simulink model "generic_IVS"  (R2024a)
settings: Solver=FixedStepDiscrete  StartTime=0.0  StopTime=inf  FixedStep=0.001  RelTol=1e-3  EnableMultiTasking=on
libraries: simulink x1, CarMaker4SL x1
(part 1 of 2)
settings Model: Creator=IPG  LastModifiedBy=User
settings SolverCC: AlgebraicLoopSolver=TrustRegion
settings DataIOCC: LimitDataPoints=on  SaveFormat=Array  SignalLoggingSaveFormat=ModelDataLogs  ReturnWorkspaceOutputs=off  SignalLoggingName=sigsOut
settings OptimizationCC: BooleanDataType=off  ReuseModelBlockBuffer=off  ExpressionDepthLimit=2147483647  InitFltsAndDblsToZero=on  LifeSpan=inf
settings DebuggingCC: SaveWithParameterizedLinksMsg=none  UnderspecifiedInitializationDetection=Classic  MergeDetectMultiDrivingBlocksExec=none  SignalResolutionControl=TryResolveAllWithWarning  MultiTaskDSMMsg=warning  MultiTaskCondExecSysMsg=none  FcnCallInpInsideContextMsg=warning  UnconnectedInputMsg=warning  UnconnectedOutputMsg=warning  UnconnectedLineMsg=warning  StateNameClashWarn=warning  SFUnexpectedBacktrackingDiag=warning  SFNoUnconditionalDefaultTransitionDiag=warning  ArithmeticOperatorsInVariantConditions=warning
settings HardwareCC: ProdBitPerPointer=32  ProdBitPerSizeT=32  ProdBitPerPtrDiffT=32  ProdLargestAtomicFloat=None  ProdIntDivRoundTo=Undefined  ProdEndianess=Unspecified  ProdWordSize=32  ProdHWDeviceType=32-bit Generic  TargetBitPerPointer=64  TargetBitPerSizeT=64  TargetBitPerPtrDiffT=64  TargetLongLongMode=on  TargetIntDivRoundTo=Zero  TargetEndianess=LittleEndian  TargetWordSize=64  TargetHWDeviceType=MATLAB Host  ProdEqTarget=off
settings ModelReferenceCC: EnableRefExpFcnMdlSchedulingChecks=on  PropagateSignalLabelsOutOfModel=off
settings SFSimCC: SimUseLocalCustomCode=off  CustomCodeUndefinedFunction=UseInterfaceOnly
settings RTWCC: RTWUseLocalCustomCode=off  GPUComputeCapability=3.5  DLArmComputeVersion=19.05
settings CodeAppCC: MaxIdLength=63  StateflowObjectComments=on
settings GRTTargetCC: TargetFcnLib=ansi_tfl_tmw.mat  TargetLangStandard=C89/C90 (ANSI)  CombineOutputUpdateFcns=off  GRTInterface=on
settings ConfigComp: CovMetricSettings=dw  CovSaveCumulativeToWorkspaceVar=on  CovSaveSingleToWorkspaceVar=on  CovExternalEMLEnable=off

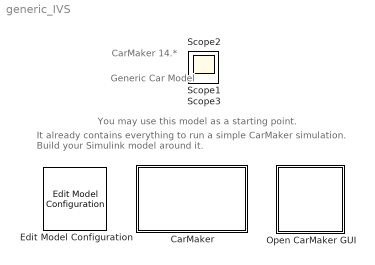
== system generic_IVS ==
  note: Generic Car Model
  note: You may use this model as a starting point.
  note: It already contains everything to run a simple CarMaker simulation.
      | Build your Simulink model around it.
  note: CarMaker 14.*
  CarMaker : Subsystem  TreatAsAtomicUnit=on
      mask Display: image(imread('CarMakerSys.png'));
  Edit Model Configuration : CarMaker4SL/Edit Model Configuration  SFunctionModules=''
  Open CarMaker GUI : Subsystem  LoadFcn=if ~length(which('cmself')), cmenv; end
      settings: OpenFcn=cmblockmagic('gui_fix_display'); CM_Simulink
      mask Display: image(imread('CarMakerGUI.png'));
  Scope1 : Scope
  Scope2 : Scope
  Scope3 : Scope

== system generic_IVS/CarMaker ==
  note: Do Not Modify !!
  note: Modify !!
  CM_FIRST : Subsystem
  CM_LAST : Subsystem
  DrivMan : Subsystem
  Ground : Ground
  IPG Vehicle : Subsystem
  Subsystem : Subsystem
  Terminator : Terminator
  VehicleControl : Subsystem
  wires:
  DrivMan/2(DrivMan.Out) -> VehicleControl/2(DrivMan.In)
  DrivMan/1(Sync_Out) -> VehicleControl/1(Sync_In)
  CM_FIRST/2(Env.Misc) -> DrivMan/2(Env.Misc)
  CM_FIRST/1(Sync_Out) -> DrivMan/1(Sync_In)
  CM_LAST/1(Sync_Out) -> Terminator/1
  Ground/1 -> CM_FIRST/1(Sync_In)
  IPG Vehicle/1(Sync_Out) -> CM_LAST/1(Sync_In)
  VehicleControl/1(Sync_Out) -> IPG Vehicle/1(Sync_In)
  VehicleControl/3(VhclCtrl.Steering) -> IPG Vehicle/3(VhclCtrl.Steering)
  VehicleControl/4(Vhcl.Wheel.In) -> IPG Vehicle/4(Vhcl.Wheel.In)
  VehicleControl/5(Vhcl.Misc) -> IPG Vehicle/5(Vhcl.Misc)
  VehicleControl/6(VhclCtrl.Brake) -> IPG Vehicle/6(VhclCtrl.Brake)
  VehicleControl/7(VhclCtrl.PT) -> IPG Vehicle/7(VhclCtrl.PT)
  VehicleControl/2(Vhcl.Model.Source) -> IPG Vehicle/2(Vhcl.Model.Source)

== system generic_IVS/Open CarMaker GUI ==
  S-Function : S-Function  FunctionName=cm_gui  SFunctionDeploymentMode=off  EnableBusSupport=off

== system generic_IVS/CarMaker/CM_FIRST ==
  Sync_In : Inport
  BusCreator1 : BusCreator  Inputs=8
  BusCreator2 : BusCreator  Inputs=6
  Demux1 : Demux  Outputs=14
      settings: DisplayOption=none
  Environment : S-Function  FunctionName=CM_Sfun  Parameters='Environment'  SFunctionDeploymentMode=off  EnableBusSupport=off
  IoIn : S-Function  FunctionName=CM_Sfun  Parameters='IoIn'  SFunctionDeploymentMode=off  EnableBusSupport=off
  Terminator : Terminator
  Sync_Out : Outport  VectorParamsAs1DForOutWhenUnconnected=off
  Env.Misc : Outport  Port=2  VectorParamsAs1DForOutWhenUnconnected=off
  wires:
  BusCreator2/1 -> Terminator/1  "IF Environment (in)"
  BusCreator1/1 -> Env.Misc/1
  Demux1/14 -> BusCreator2/6  "Env sRoad"
  Demux1/13 -> BusCreator2/5  "Env PoI_GCS Elev"
  Demux1/12 -> BusCreator2/4  "Env PoI_GCS Lat"
  Demux1/11 -> BusCreator2/3  "Env PoI_GCS Long"
  Demux1/10 -> BusCreator2/2  "Env Time"
  Demux1/9 -> BusCreator2/1  "Env yDay"
  Demux1/8 -> BusCreator1/8  "Env WindVel_tot z"
  Demux1/7 -> BusCreator1/7  "Env WindVel_tot y"
  Demux1/6 -> BusCreator1/6  "Env WindVel_tot x"
  Demux1/5 -> BusCreator1/5  "Env SolarRadiation"
  Demux1/4 -> BusCreator1/4  "Env AirHumidity"
  Demux1/3 -> BusCreator1/3  "Env AirPressure"
  Demux1/2 -> BusCreator1/2  "Env AirDensity"
  Demux1/1 -> BusCreator1/1  "Env Temperature"
  Environment/2 -> Demux1/1
  Environment/1 -> Sync_Out/1
  IoIn/1 -> Environment/1
  Sync_In/1 -> IoIn/1

== system generic_IVS/CarMaker/CM_LAST ==
  Sync_In : Inport
  CM_User : S-Function  FunctionName=CM_Sfun  Parameters='CM_User'  SFunctionDeploymentMode=off  EnableBusSupport=off
  IoOut : S-Function  FunctionName=CM_Sfun  Parameters='IoOut'  SFunctionDeploymentMode=off  EnableBusSupport=off
  Sync_Out : Outport  VectorParamsAs1DForOutWhenUnconnected=off
  wires:
  IoOut/1 -> Sync_Out/1
  CM_User/1 -> IoOut/1
  Sync_In/1 -> CM_User/1

== system generic_IVS/CarMaker/DrivMan ==
  note: There's rarely a reason to override DrivMan signals.
      | Use the VehicleControl interface for this purpose.
  Sync_In : Inport
  Env.Misc : Inport  Port=2
  BusCreator : BusCreator  Inputs=20
  Demux : Demux  Outputs=20
      settings: DisplayOption=none
  DrivMan : S-Function  FunctionName=CM_Sfun  Parameters='DrivMan'  SFunctionDeploymentMode=off  EnableBusSupport=off
  Sync_Out : Outport  VectorParamsAs1DForOutWhenUnconnected=off
  DrivMan.Out : Outport  Port=2  VectorParamsAs1DForOutWhenUnconnected=off
  wires:
  Demux/8 -> BusCreator/8  "DrivMan SelectorCtrl"
  Demux/7 -> BusCreator/7  "DrivMan UserSignal4"
  Demux/6 -> BusCreator/6  "DrivMan UserSignal3"
  Demux/5 -> BusCreator/5  "DrivMan UserSignal2"
  Demux/4 -> BusCreator/4  "DrivMan UserSignal1"
  Demux/3 -> BusCreator/3  "DrivMan UserSignal0"
  Demux/2 -> BusCreator/2  "DrivMan Key"
  Demux/1 -> BusCreator/1  "DrivMan SST"
  Env.Misc/1 -> DrivMan/2
  Sync_In/1 -> DrivMan/1
  DrivMan/1 -> Sync_Out/1
  BusCreator/1 -> DrivMan.Out/1
  DrivMan/2 -> Demux/1
  Demux/9 -> BusCreator/9  "DrivMan DigitalSelectorCtrl0"
  Demux/10 -> BusCreator/10  "DrivMan DigitalSelectorCtrl1"
  Demux/11 -> BusCreator/11  "DrivMan DigitalSelectorCtrl2"
  Demux/20 -> BusCreator/20  "DrivMan Steering Trq"
  Demux/19 -> BusCreator/19  "DrivMan Steering AngAcc"
  Demux/18 -> BusCreator/18  "DrivMan Steering AngVel"
  Demux/17 -> BusCreator/17  "DrivMan Steering Ang"
  Demux/16 -> BusCreator/16  "DrivMan Gas"
  Demux/15 -> BusCreator/15  "DrivMan Clutch"
  Demux/14 -> BusCreator/14  "DrivMan BrakePark"
  Demux/13 -> BusCreator/13  "DrivMan Brake"
  Demux/12 -> BusCreator/12  "DrivMan GearNo"

== system generic_IVS/CarMaker/IPG Vehicle ==
  Sync_In : Inport
  Vhcl.Model.Source : Inport  Port=2
  VhclCtrl.Steering : Inport  Port=3
  Vhcl.Wheel.In : Inport  Port=4
  Vhcl.Misc : Inport  Port=5
  VhclCtrl.Brake : Inport  Port=6
  VhclCtrl.PT : Inport  Port=7
  Brake : Subsystem
  CarAndTrailer : Subsystem
  PowerTrain : Subsystem
  Stop Simulation : Stop
  VehicleSource_BuiltIn : simulink/Logic and Bit Operations/Compare To Constant  relop=~=  const=1  OutDataTypeStr=boolean  ZeroCross=off
  Sync_Out : Outport  VectorParamsAs1DForOutWhenUnconnected=off
  wires:
  VhclCtrl.PT/1 -> PowerTrain/3(VhclCtrl.PT)
  Brake/1(Sync_Out) -> PowerTrain/1(Sync_In)
  CarAndTrailer/1(Sync_Out) -> Brake/1(Sync_In)
  CarAndTrailer/2(Brake.IF.In) -> Brake/2(Brake.IF.In)
  VhclCtrl.Brake/1 -> Brake/3(VhclCtrl.Brake)
  PowerTrain/1(Sync_Out) -> Sync_Out/1
  Vhcl.Misc/1 -> CarAndTrailer/4(Vhcl.Misc)
  Vhcl.Wheel.In/1 -> CarAndTrailer/3(Vhcl.Wheel.In)
  VhclCtrl.Steering/1 -> CarAndTrailer/2(VhclCtrl.Steering)
  Sync_In/1 -> CarAndTrailer/1(Sync_In)
  Vhcl.Model.Source/1 -> VehicleSource_BuiltIn/1
  VehicleSource_BuiltIn/1 -> Stop Simulation/1
  Brake/2(Vhcl.Wheel.PT) -> PowerTrain/2(Vhcl.Wheel.PT)

== system generic_IVS/CarMaker/Subsystem ==
  Day1 : Subsystem  Commented=on
  Day2 : Subsystem  Commented=on
  Day3 : Subsystem  Commented=on
  Day4 & 5 : Subsystem  Commented=on
  Day6 : Subsystem  Commented=on
  Final Project : Subsystem

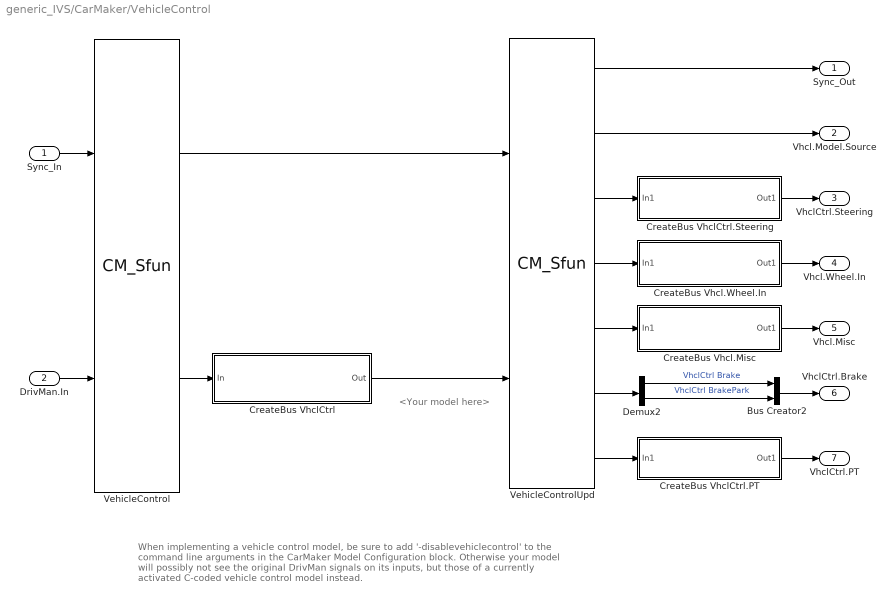
== system generic_IVS/CarMaker/VehicleControl ==
  note: <Your model here>
  note: When implementing a vehicle control model,
      | be sure to add '-disablevehiclecontrol' to the command line arguments
      | in the CarMaker Model Configuration block.
      | Otherwise your model will possibly not see the original DrivMan signals
      | on its inputs, but those of a currently activated C-coded vehicle control model instead.
  Sync_In : Inport
  DrivMan.In : Inport  Port=2
  Bus Creator2 : BusCreator  Inputs=2
  CreateBus Vhcl.Misc : Subsystem
  CreateBus Vhcl.Wheel.In : Subsystem
  CreateBus VhclCtrl : Subsystem
  CreateBus VhclCtrl.PT : Subsystem
  CreateBus VhclCtrl.Steering : Subsystem
  Demux2 : Demux  Outputs=2
      settings: DisplayOption=none
  VehicleControl : S-Function  FunctionName=CM_Sfun  Parameters='VehicleControl'  SFunctionDeploymentMode=off  EnableBusSupport=off
  VehicleControlUpd : S-Function  FunctionName=CM_Sfun  Parameters='VehicleControlUpd'  SFunctionDeploymentMode=off  EnableBusSupport=off
  Sync_Out : Outport  VectorParamsAs1DForOutWhenUnconnected=off
  Vhcl.Model.Source : Outport  Port=2  VectorParamsAs1DForOutWhenUnconnected=off
  VhclCtrl.Steering : Outport  Port=3  VectorParamsAs1DForOutWhenUnconnected=off
  Vhcl.Wheel.In : Outport  Port=4  VectorParamsAs1DForOutWhenUnconnected=off
  Vhcl.Misc : Outport  Port=5  VectorParamsAs1DForOutWhenUnconnected=off
  VhclCtrl.Brake : Outport  Port=6  VectorParamsAs1DForOutWhenUnconnected=off
  VhclCtrl.PT : Outport  Port=7  VectorParamsAs1DForOutWhenUnconnected=off
  wires:
  CreateBus VhclCtrl/1(Out) -> VehicleControlUpd/2
  VehicleControl/2 -> CreateBus VhclCtrl/1(In)
  VehicleControlUpd/2 -> Vhcl.Model.Source/1
  VehicleControlUpd/4 -> CreateBus Vhcl.Wheel.In/1(In1)
  VehicleControlUpd/5 -> CreateBus Vhcl.Misc/1(In1)
  VehicleControlUpd/6 -> Demux2/1
  VehicleControlUpd/7 -> CreateBus VhclCtrl.PT/1(In1)
  VehicleControlUpd/3 -> CreateBus VhclCtrl.Steering/1(In1)
  CreateBus Vhcl.Misc/1(Out1) -> Vhcl.Misc/1
  CreateBus Vhcl.Wheel.In/1(Out1) -> Vhcl.Wheel.In/1
  DrivMan.In/1 -> VehicleControl/2
  VehicleControl/1 -> VehicleControlUpd/1
  Sync_In/1 -> VehicleControl/1
  CreateBus VhclCtrl.PT/1(Out1) -> VhclCtrl.PT/1
  Bus Creator2/1 -> VhclCtrl.Brake/1
  CreateBus VhclCtrl.Steering/1(Out1) -> VhclCtrl.Steering/1
  VehicleControlUpd/1 -> Sync_Out/1
  Demux2/2 -> Bus Creator2/2  "VhclCtrl BrakePark"
  Demux2/1 -> Bus Creator2/1  "VhclCtrl Brake"

== system generic_IVS/CarMaker/IPG Vehicle/Brake ==
  note: When replacing the entire braking system,
      | be sure to disable the IPG brake model by using the brake
      | model 'Model Manager off' in the vehicle GUI.
  note: <Your model here>
  Sync_In : Inport
  Brake.IF.In : Inport  Port=2
  VhclCtrl.Brake : Inport  Port=3
  Brake : S-Function  FunctionName=CM_Sfun  Parameters='Brake'  SFunctionDeploymentMode=off  EnableBusSupport=off
  BrakeUpd : S-Function  FunctionName=CM_Sfun  Parameters='BrakeUpd'  SFunctionDeploymentMode=off  EnableBusSupport=off
  BusCreator1 : BusCreator  Inputs=16
  CreateBus Vhcl.Wheel.PT : Subsystem
  Demux : Demux  Outputs=16
      settings: DisplayOption=none
  Sync_Out : Outport  VectorParamsAs1DForOutWhenUnconnected=off
  Vhcl.Wheel.PT : Outport  Port=2  VectorParamsAs1DForOutWhenUnconnected=off
  wires:
  Demux/16 -> BusCreator1/16  "Brake IF Trq_DriveSrc_trg d3"
  Demux/15 -> BusCreator1/15  "Brake IF Trq_DriveSrc_trg d2"
  Demux/14 -> BusCreator1/14  "Brake IF Trq_DriveSrc_trg d1"
  Demux/13 -> BusCreator1/13  "Brake IF Trq_DriveSrc_trg d0"
  Demux/12 -> BusCreator1/12  "Brake IF Trq_Reg_trg RR"
  Demux/11 -> BusCreator1/11  "Brake IF Trq_Reg_trg RL"
  Demux/10 -> BusCreator1/10  "Brake IF Trq_Reg_trg FR"
  Demux/9 -> BusCreator1/9  "Brake IF Trq_Reg_trg FL"
  Demux/8 -> BusCreator1/8  "Brake IF Trq_PB RR"
  Demux/7 -> BusCreator1/7  "Brake IF Trq_PB RL"
  Demux/6 -> BusCreator1/6  "Brake IF Trq_PB FR"
  Demux/5 -> BusCreator1/5  "Brake IF Trq_PB FL"
  Demux/4 -> BusCreator1/4  "Brake IF Trq_WB RR"
  Demux/3 -> BusCreator1/3  "Brake IF Trq_WB RL"
  Demux/2 -> BusCreator1/2  "Brake IF Trq_WB FR"
  Demux/1 -> BusCreator1/1  "Brake IF Trq_WB FL"
  Brake/2 -> Demux/1
  BusCreator1/1 -> BrakeUpd/2
  BrakeUpd/1 -> Sync_Out/1
  Brake/1 -> BrakeUpd/1  "Sync"
  Brake.IF.In/1 -> Brake/2
  VhclCtrl.Brake/1 -> Brake/3
  Sync_In/1 -> Brake/1
  BrakeUpd/2 -> CreateBus Vhcl.Wheel.PT/1(In)
  CreateBus Vhcl.Wheel.PT/1(Out) -> Vhcl.Wheel.PT/1

== system generic_IVS/CarMaker/IPG Vehicle/CarAndTrailer ==
  Sync_In : Inport
  VhclCtrl.Steering : Inport  Port=2
  Vhcl.Wheel.In : Inport  Port=3
  Vhcl.Misc : Inport  Port=4
  CarAndTrailerUpd : Subsystem
  Forces : Subsystem
  Ground : Ground
  Kinematics : Subsystem
  Kinetics : Subsystem
  Steering : Subsystem
  Terminator : Terminator
  Terminator1 : Terminator
  Trailer : Subsystem
  Sync_Out : Outport  VectorParamsAs1DForOutWhenUnconnected=off
  Brake.IF.In : Outport  Port=2  VectorParamsAs1DForOutWhenUnconnected=off
  wires:
  Trailer/9(Car.Hitch.FrcTrq) -> CarAndTrailerUpd/9(Car.Hitch.FrcTrq)
  Trailer/8(Vhcl.Wheel.RR) -> CarAndTrailerUpd/8(Vhcl.Wheel.RR)
  Trailer/7(Vhcl.Wheel.RL) -> CarAndTrailerUpd/7(Vhcl.Wheel.RL)
  Trailer/6(Vhcl.Wheel.FR) -> CarAndTrailerUpd/6(Vhcl.Wheel.FR)
  Trailer/5(Vhcl.Wheel.FL) -> CarAndTrailerUpd/5(Vhcl.Wheel.FL)
  Trailer/4(Vhcl.PoI) -> CarAndTrailerUpd/4(Vhcl.PoI)
  Trailer/3(Vhcl.Motion) -> CarAndTrailerUpd/3(Vhcl.Motion)
  Trailer/2(Vhcl.Steering) -> CarAndTrailerUpd/2(Vhcl.Steering)
  Trailer/1(Sync_Out) -> CarAndTrailerUpd/1(Sync_In)
  CarAndTrailerUpd/2(Brake.IF.In) -> Brake.IF.In/1
  CarAndTrailerUpd/1(Sync_Out) -> Sync_Out/1
  Vhcl.Misc/1 -> Terminator1/1
  Vhcl.Wheel.In/1 -> Terminator/1
  Kinetics/6(WheelCarrier.Misc) -> Trailer/6(WheelCarrier.Misc)
  Kinetics/5(Car.Trq_T2W) -> Trailer/5(Car.Trq_T2W)
  Steering/2(Steer.IF) -> Kinematics/2(Steer.IF)
  Kinetics/4(Car.Fr1) -> Trailer/4(Car.Fr1)
  Kinetics/3(Car.Hitch) -> Trailer/3(Car.Hitch)
  Kinetics/2(Trailer.Load) -> Trailer/2(Trailer.Load)
  VhclCtrl.Steering/1 -> Steering/2(VhclCtrl.Steering)
  Sync_In/1 -> Steering/1(Sync_In)
  Steering/1(Sync_Out) -> Kinematics/1(Sync_In)
  Kinetics/1(Sync_Out) -> Trailer/1(Sync_In)
  Ground/1 -> CarAndTrailerUpd/10(Vhcl.Fr1A)
  Forces/8(TireRR_Out) -> Kinetics/8(TireRR.Out)
  Forces/7(TireRL_Out) -> Kinetics/7(TireRL.Out)
  Forces/6(TireFR_Out) -> Kinetics/6(TireFR.Out)
  Forces/5(TireFL_Out) -> Kinetics/5(TireFL.Out)
  Forces/4(Car.Load) -> Kinetics/4(Car.Load)
  Forces/2(Car.Virtual) -> Kinetics/2(Car.Virtual)
  Kinematics/6(lSpring) -> Forces/6(lSpring)
  Kinematics/7(vDamp) -> Forces/7(vDamp)
  Forces/3(Car.Aero) -> Kinetics/3(Car.Aero)
  Forces/1(Sync_Out) -> Kinetics/1(Sync_In)
  Kinematics/5(TireRR_In) -> Forces/5(TireRR_In)
  Kinematics/4(TireRL_In) -> Forces/4(TireRL_In)
  Kinematics/3(TireFR_In) -> Forces/3(TireFR_In)
  Kinematics/2(TireFL_In) -> Forces/2(TireFL_In)
  Kinematics/1(Sync_Out) -> Forces/1(Sync_In)
  Kinematics/8(lStabi) -> Forces/8(lStabi)
  Kinematics/9(lBuf) -> Forces/9(lBuf)

== system generic_IVS/CarMaker/IPG Vehicle/PowerTrain ==
  note: When replacing the entire powertrain,
      | be sure to disable the IPG powertrain model by using the powertrain
      | model 'Model Manager off' in the vehicle GUI.
  note: <Your model here>
  Sync_In : Inport
  Vhcl.Wheel.PT : Inport  Port=2
  VhclCtrl.PT : Inport  Port=3
  BusCreator1 : BusCreator  Inputs=42
  Demux1 : Demux  Outputs=42
      settings: DisplayOption=none
  PowerTrain : S-Function  FunctionName=CM_Sfun  Parameters='PowerTrain'  SFunctionDeploymentMode=off  EnableBusSupport=off
  PowerTrainUpd : S-Function  FunctionName=CM_Sfun  Parameters='PowerTrainUpd'  SFunctionDeploymentMode=off  EnableBusSupport=off
  Sync_Out : Outport  VectorParamsAs1DForOutWhenUnconnected=off
  wires:
  BusCreator1/1 -> PowerTrainUpd/2
  Demux1/42 -> BusCreator1/42  "PT IF WRR Trq_BrakeReg_max"
  Demux1/41 -> BusCreator1/41  "PT IF WRR Trq_BrakeReg"
  Demux1/40 -> BusCreator1/40  "PT IF WRR Trq_Supp2WC"
  Demux1/39 -> BusCreator1/39  "PT IF WRR Trq_Drive"
  Demux1/38 -> BusCreator1/38  "PT IF WRR Trq_B2W"
  Demux1/37 -> BusCreator1/37  "PT IF WRR rotv"
  Demux1/36 -> BusCreator1/36  "PT IF WRR rot"
  Demux1/35 -> BusCreator1/35  "PT IF WRL Trq_BrakeReg_max"
  Demux1/34 -> BusCreator1/34  "PT IF WRL Trq_BrakeReg"
  Demux1/33 -> BusCreator1/33  "PT IF WRL Trq_Supp2WC"
  Demux1/32 -> BusCreator1/32  "PT IF WRL Trq_Drive"
  Demux1/31 -> BusCreator1/31  "PT IF WRL Trq_B2W"
  Demux1/30 -> BusCreator1/30  "PT IF WRL rotv"
  Demux1/29 -> BusCreator1/29  "PT IF WRL rot"
  Demux1/28 -> BusCreator1/28  "PT IF WFR Trq_BrakeReg_max"
  Demux1/27 -> BusCreator1/27  "PT IF WFR Trq_BrakeReg"
  Demux1/26 -> BusCreator1/26  "PT IF WFR Trq_Supp2WC"
  Demux1/25 -> BusCreator1/25  "PT IF WFR Trq_Drive"
  Demux1/24 -> BusCreator1/24  "PT IF WFR Trq_B2W"
  Demux1/23 -> BusCreator1/23  "PT IF WFR rotv"
  Demux1/22 -> BusCreator1/22  "PT IF WFR rot"
  Demux1/21 -> BusCreator1/21  "PT IF WFL Trq_BrakeReg_max"
  Demux1/20 -> BusCreator1/20  "PT IF WFL Trq_BrakeReg"
  Demux1/19 -> BusCreator1/19  "PT IF WFL Trq_Supp2WC"
  Demux1/18 -> BusCreator1/18  "PT IF WFL Trq_Drive"
  Demux1/17 -> BusCreator1/17  "PT IF WFL Trq_B2W"
  Demux1/16 -> BusCreator1/16  "PT IF WFL rotv"
  Demux1/15 -> BusCreator1/15  "PT IF WFL rot"
  Demux1/14 -> BusCreator1/14  "PT IF DL_iDiff_mean"
  Demux1/13 -> BusCreator1/13  "PT IF Trq_Supp2BdyEng y"
  Demux1/12 -> BusCreator1/12  "PT IF Trq_Supp2BdyEng x"
  Demux1/11 -> BusCreator1/11  "PT IF Trq_Supp2Bdy1B z"
  Demux1/10 -> BusCreator1/10  "PT IF Trq_Supp2Bdy1B y"
  Demux1/9 -> BusCreator1/9  "PT IF Trq_Supp2Bdy1B x"
  Demux1/8 -> BusCreator1/8  "PT IF Trq_Supp2Bdy1 z"
  Demux1/7 -> BusCreator1/7  "PT IF Trq_Supp2Bdy1 y"
  Demux1/6 -> BusCreator1/6  "PT IF Trq_Supp2Bdy1 x"
  Demux1/5 -> BusCreator1/5  "PT IF Engine_rotv"
  Demux1/4 -> BusCreator1/4  "PT IF GearNo"
  Demux1/3 -> BusCreator1/3  "PT IF OperationError"
  Demux1/2 -> BusCreator1/2  "PT IF OperationState"
  Demux1/1 -> BusCreator1/1  "PT IF Ignition"
  Sync_In/1 -> PowerTrain/1
  PowerTrain/2 -> Demux1/1
  PowerTrainUpd/1 -> Sync_Out/1
  PowerTrain/1 -> PowerTrainUpd/1  "Sync"
  VhclCtrl.PT/1 -> PowerTrain/3
  Vhcl.Wheel.PT/1 -> PowerTrain/2

== system generic_IVS/CarMaker/Subsystem/Day1 ==
  Scenario 1 : Subsystem  Commented=on  ReferencedSubsystem=Day1_Scenario_1
  Scenario 2 : Subsystem  Commented=on  ReferencedSubsystem=Day1_Scenario_2
  Scenario 3 & 4 : Subsystem  Commented=on  ReferencedSubsystem=Day1_Scenario_3_4

== system generic_IVS/CarMaker/Subsystem/Day2 ==
  Scenario 1 : Subsystem  ReferencedSubsystem=Day2_Scenario_1
  Scenario 2 & 3 : Subsystem  ReferencedSubsystem=Day2_Scenario_2_3
  Scenario 4 & 5 : Subsystem  ReferencedSubsystem=Day2_Scenario_4_5

== system generic_IVS/CarMaker/Subsystem/Day3 ==
  note: Do Not Modify !!
  Chart : Stateflow chart  TreatAsAtomicUnit=on
  Function-Call Split : FunctionCallSplit  IconShape=distinctive  NumOutputPorts=2  OutputPortLayout=default
  Scenario 1 : Subsystem  TreatAsAtomicUnit=on  ReferencedSubsystem=Day3_Scenario_1
  Scenario 2 : Subsystem  TreatAsAtomicUnit=on  ReferencedSubsystem=Day3_Scenario_2
  wires:
  Chart/1(do_Logic()) -> Function-Call Split/1
  [do_Logic] -> Scenario 1/Trigger
  [do_Logic_] -> Scenario 2/Trigger
  Function-Call Split/1 -> [do_Logic]
  Function-Call Split/2 -> [do_Logic_]

== system generic_IVS/CarMaker/Subsystem/Day4 & 5 ==
  Scenario 1 : Subsystem  ReferencedSubsystem=Day4_5_Scenario_1

== system generic_IVS/CarMaker/Subsystem/Day6 ==
  Scenario 1 : Subsystem  ReferencedSubsystem=Day6_Scenario_1

== system generic_IVS/CarMaker/Subsystem/Final Project ==
  Scenario 1 : Subsystem  ReferencedSubsystem=Final_Project

== system generic_IVS/CarMaker/VehicleControl/CreateBus Vhcl.Misc ==
  In1 : Inport
  BusCreator : BusCreator  Inputs=11
  Demux : Demux  Outputs=11
      settings: DisplayOption=none
  Out1 : Outport  VectorParamsAs1DForOutWhenUnconnected=off
  wires:
  Demux/11 -> BusCreator/11  "Vhcl Wind_vel_0 z"
  Demux/10 -> BusCreator/10  "Vhcl Wind_vel_0 y"
  Demux/9 -> BusCreator/9  "Vhcl Wind_vel_0 x"
  Demux/8 -> BusCreator/8  "Vhcl Trq_DL2BdyEng y"
  Demux/7 -> BusCreator/7  "Vhcl Trq_DL2BdyEng x"
  Demux/6 -> BusCreator/6  "Vhcl Trq_DL2Bdy1B z"
  Demux/5 -> BusCreator/5  "Vhcl Trq_DL2Bdy1B y"
  Demux/4 -> BusCreator/4  "Vhcl Trq_DL2Bdy1B x"
  Demux/3 -> BusCreator/3  "Vhcl Trq_DL2Bdy1 z"
  Demux/2 -> BusCreator/2  "Vhcl Trq_DL2Bdy1 y"
  Demux/1 -> BusCreator/1  "Vhcl Trq_DL2Bdy1 x"
  In1/1 -> Demux/1
  BusCreator/1 -> Out1/1

== system generic_IVS/CarMaker/VehicleControl/CreateBus Vhcl.Wheel.In ==
  In1 : Inport
  Bus Creator1 : BusCreator  Inputs=12
  Demux1 : Demux  Outputs=12
      settings: DisplayOption=none
  Out1 : Outport  VectorParamsAs1DForOutWhenUnconnected=off
  wires:
  Demux1/12 -> Bus Creator1/12  "Vhcl Wheel RR rotv"
  Demux1/11 -> Bus Creator1/11  "Vhcl Wheel RR Trq_DL2WC"
  Demux1/10 -> Bus Creator1/10  "Vhcl Wheel RR Trq_B2WC"
  Demux1/9 -> Bus Creator1/9  "Vhcl Wheel RL rotv"
  Demux1/8 -> Bus Creator1/8  "Vhcl Wheel RL Trq_DL2WC"
  Demux1/7 -> Bus Creator1/7  "Vhcl Wheel RL Trq_B2WC"
  Demux1/6 -> Bus Creator1/6  "Vhcl Wheel FR rotv"
  Demux1/5 -> Bus Creator1/5  "Vhcl Wheel FR Trq_DL2WC"
  Demux1/4 -> Bus Creator1/4  "Vhcl Wheel FR Trq_B2WC"
  Demux1/3 -> Bus Creator1/3  "Vhcl Wheel FL rotv"
  In1/1 -> Demux1/1
  Bus Creator1/1 -> Out1/1
  Demux1/2 -> Bus Creator1/2  "Vhcl Wheel FL Trq_DL2WC"
  Demux1/1 -> Bus Creator1/1  "Vhcl Wheel FL Trq_B2WC"

== system generic_IVS/CarMaker/VehicleControl/CreateBus VhclCtrl ==
  In : Inport
  BusCreator : BusCreator  Inputs=29
  Demux : Demux  Outputs=29
      settings: DisplayOption=none
  Out : Outport  VectorParamsAs1DForOutWhenUnconnected=off
  wires:
  In/1 -> Demux/1
  BusCreator/1 -> Out/1
  Demux/1 -> BusCreator/1  "VhclCtrl SST"
  Demux/2 -> BusCreator/2  "VhclCtrl Key"
  Demux/3 -> BusCreator/3  "VhclCtrl UserSignal0"
  Demux/4 -> BusCreator/4  "VhclCtrl UserSignal1"
  Demux/5 -> BusCreator/5  "VhclCtrl UserSignal2"
  Demux/6 -> BusCreator/6  "VhclCtrl UserSignal3"
  Demux/7 -> BusCreator/7  "VhclCtrl UserSignal4"
  Demux/8 -> BusCreator/8  "VhclCtrl GearNo"
  Demux/9 -> BusCreator/9  "VhclCtrl SelectorCtrl"
  Demux/10 -> BusCreator/10  "VhclCtrl Brake"
  Demux/11 -> BusCreator/11  "VhclCtrl BrakePark"
  Demux/12 -> BusCreator/12  "VhclCtrl Clutch"
  Demux/13 -> BusCreator/13  "VhclCtrl Gas"
  Demux/14 -> BusCreator/14  "VhclCtrl Steering Ang"
  Demux/15 -> BusCreator/15  "VhclCtrl Steering AngVel"
  Demux/16 -> BusCreator/16  "VhclCtrl Steering AngAcc"
  Demux/17 -> BusCreator/17  "VhclCtrl Steering Trq"
  Demux/18 -> BusCreator/18  "VhclCtrl Lights LowBeam"
  Demux/19 -> BusCreator/19  "VhclCtrl Lights HighBeam"
  Demux/20 -> BusCreator/20  "VhclCtrl Lights Daytime"
  Demux/21 -> BusCreator/21  "VhclCtrl Lights ParkL"
  Demux/22 -> BusCreator/22  "VhclCtrl Lights ParkR"
  Demux/23 -> BusCreator/23  "VhclCtrl Lights IndL"
  Demux/24 -> BusCreator/24  "VhclCtrl Lights IndR"
  Demux/25 -> BusCreator/25  "VhclCtrl Lights FogFrontL"
  Demux/26 -> BusCreator/26  "VhclCtrl Lights FogFrontR"
  Demux/27 -> BusCreator/27  "VhclCtrl Lights FogRear"
  Demux/28 -> BusCreator/28  "VhclCtrl Lights Brake"
  Demux/29 -> BusCreator/29  "VhclCtrl Lights Reverse"

== system generic_IVS/CarMaker/VehicleControl/CreateBus VhclCtrl.PT ==
  In1 : Inport
  BusCreator1 : BusCreator  Inputs=12
  Demux1 : Demux  Outputs=12
      settings: DisplayOption=none
  Out1 : Outport  VectorParamsAs1DForOutWhenUnconnected=off
  wires:
  Demux1/12 -> BusCreator1/12  "VhclCtrl Brake"
  Demux1/11 -> BusCreator1/11  "VhclCtrl Gas"
  Demux1/10 -> BusCreator1/10  "VhclCtrl Clutch"
  Demux1/9 -> BusCreator1/9  "VhclCtrl SelectorCtrl"
  Demux1/8 -> BusCreator1/8  "VhclCtrl GearNo"
  Demux1/7 -> BusCreator1/7  "VhclCtrl UserSignal4"
  Demux1/6 -> BusCreator1/6  "VhclCtrl UserSignal3"
  Demux1/5 -> BusCreator1/5  "VhclCtrl UserSignal2"
  Demux1/4 -> BusCreator1/4  "VhclCtrl UserSignal1"
  Demux1/3 -> BusCreator1/3  "VhclCtrl UserSignal0"
  Demux1/2 -> BusCreator1/2  "VhclCtrl Key"
  Demux1/1 -> BusCreator1/1  "VhclCtrl SST"
  In1/1 -> Demux1/1
  BusCreator1/1 -> Out1/1

== system generic_IVS/CarMaker/VehicleControl/CreateBus VhclCtrl.Steering ==
  In1 : Inport
  Bus Creator : BusCreator  Inputs=5
  Demux : Demux  Outputs=5
      settings: DisplayOption=none
  Out1 : Outport  VectorParamsAs1DForOutWhenUnconnected=off
  wires:
  In1/1 -> Demux/1
  Bus Creator/1 -> Out1/1
  Demux/1 -> Bus Creator/1  "VhclCtrl Steering Ang"
  Demux/5 -> Bus Creator/5  "VhclCtrl Steering SteerByTrq"
  Demux/3 -> Bus Creator/3  "VhclCtrl Steering AngAcc"
  Demux/2 -> Bus Creator/2  "VhclCtrl Steering AngVel"
  Demux/4 -> Bus Creator/4  "VhclCtrl Steering Trq"

== system generic_IVS/CarMaker/IPG Vehicle/Brake/CreateBus Vhcl.Wheel.PT ==
  In : Inport
  BusCreator1 : BusCreator  Inputs=20
  Demux1 : Demux  Outputs=20
      settings: DisplayOption=none
  Out : Outport  VectorParamsAs1DForOutWhenUnconnected=off
  wires:
  Demux1/20 -> BusCreator1/20  "Vhcl Trq_DriveSrc_trg d3"
  Demux1/19 -> BusCreator1/19  "Vhcl Trq_DriveSrc_trg d2"
  Demux1/18 -> BusCreator1/18  "Vhcl Trq_DriveSrc_trg d1"
  Demux1/17 -> BusCreator1/17  "Vhcl Trq_DriveSrc_trg d0"
  Demux1/16 -> BusCreator1/16  "Vhcl Wheel RR WhlBearing"
  Demux1/15 -> BusCreator1/15  "Vhcl Wheel RR Trq_T2W"
  Demux1/14 -> BusCreator1/14  "Vhcl Wheel RR Trq_BrakeReg_trg"
  Demux1/13 -> BusCreator1/13  "Vhcl Wheel RR Trq_Brake"
  Demux1/12 -> BusCreator1/12  "Vhcl Wheel RL WhlBearing"
  Demux1/11 -> BusCreator1/11  "Vhcl Wheel RL Trq_T2W"
  Demux1/10 -> BusCreator1/10  "Vhcl Wheel RL Trq_BrakeReg_trg"
  Demux1/9 -> BusCreator1/9  "Vhcl Wheel RL Trq_Brake"
  Demux1/8 -> BusCreator1/8  "Vhcl Wheel FR WhlBearing"
  Demux1/7 -> BusCreator1/7  "Vhcl Wheel FR Trq_T2W"
  Demux1/6 -> BusCreator1/6  "Vhcl Wheel FR Trq_BrakeReg_trg"
  Demux1/5 -> BusCreator1/5  "Vhcl Wheel FR Trq_Brake"
  Demux1/4 -> BusCreator1/4  "Vhcl Wheel FL WhlBearing"
  Demux1/3 -> BusCreator1/3  "Vhcl Wheel FL Trq_T2W"
  Demux1/2 -> BusCreator1/2  "Vhcl Wheel FL Trq_BrakeReg_trg"
  Demux1/1 -> BusCreator1/1  "Vhcl Wheel FL Trq_Brake"
  BusCreator1/1 -> Out/1
  In/1 -> Demux1/1

== system generic_IVS/CarMaker/IPG Vehicle/CarAndTrailer/CarAndTrailerUpd ==
  Sync_In : Inport
  Vhcl.Steering : Inport  Port=2
  Vhcl.Motion : Inport  Port=3
  Vhcl.PoI : Inport  Port=4
  Vhcl.Wheel.FL : Inport  Port=5
  Vhcl.Wheel.FR : Inport  Port=6
  Vhcl.Wheel.RL : Inport  Port=7
  Vhcl.Wheel.RR : Inport  Port=8
  Car.Hitch.FrcTrq : Inport  Port=9
  Vhcl.Fr1A : Inport  Port=10
  CarAndTrailerUpd : S-Function  FunctionName=CM_Sfun  Parameters='CarAndTrUpd'  SFunctionDeploymentMode=off  EnableBusSupport=off
  CreateBus Brake.IF.In : Subsystem
  Sync_Out : Outport  VectorParamsAs1DForOutWhenUnconnected=off
  Brake.IF.In : Outport  Port=2  VectorParamsAs1DForOutWhenUnconnected=off
  wires:
  Vhcl.Fr1A/1 -> CarAndTrailerUpd/10  "user vehicle only"
  Vhcl.Steering/1 -> CarAndTrailerUpd/2
  Vhcl.Motion/1 -> CarAndTrailerUpd/3
  Vhcl.PoI/1 -> CarAndTrailerUpd/4
  Vhcl.Wheel.FL/1 -> CarAndTrailerUpd/5
  Vhcl.Wheel.FR/1 -> CarAndTrailerUpd/6
  Car.Hitch.FrcTrq/1 -> CarAndTrailerUpd/9
  Vhcl.Wheel.RR/1 -> CarAndTrailerUpd/8
  Vhcl.Wheel.RL/1 -> CarAndTrailerUpd/7
  CarAndTrailerUpd/2 -> CreateBus Brake.IF.In/1(In)
  CreateBus Brake.IF.In/1(Out) -> Brake.IF.In/1
  CarAndTrailerUpd/1 -> Sync_Out/1
  Sync_In/1 -> CarAndTrailerUpd/1

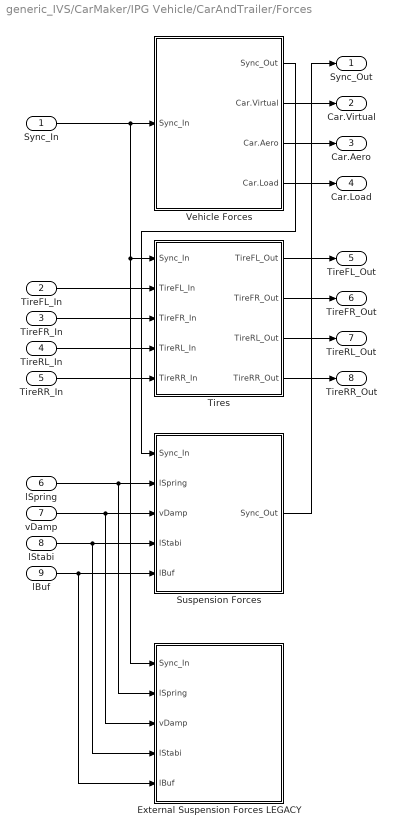
== system generic_IVS/CarMaker/IPG Vehicle/CarAndTrailer/Forces ==
  Sync_In : Inport
  TireFL_In : Inport  Port=2
  TireFR_In : Inport  Port=3
  TireRL_In : Inport  Port=4
  TireRR_In : Inport  Port=5
  lSpring : Inport  Port=6
  vDamp : Inport  Port=7
  lStabi : Inport  Port=8
  lBuf : Inport  Port=9
  External Suspension Forces LEGACY : Subsystem
  Suspension Forces : Subsystem
  Tires : Subsystem
  Vehicle Forces : Subsystem
  Sync_Out : Outport  VectorParamsAs1DForOutWhenUnconnected=off
  Car.Virtual : Outport  Port=2  VectorParamsAs1DForOutWhenUnconnected=off
  Car.Aero : Outport  Port=3  VectorParamsAs1DForOutWhenUnconnected=off
  Car.Load : Outport  Port=4  VectorParamsAs1DForOutWhenUnconnected=off
  TireFL_Out : Outport  Port=5  VectorParamsAs1DForOutWhenUnconnected=off
  TireFR_Out : Outport  Port=6  VectorParamsAs1DForOutWhenUnconnected=off
  TireRL_Out : Outport  Port=7  VectorParamsAs1DForOutWhenUnconnected=off
  TireRR_Out : Outport  Port=8  VectorParamsAs1DForOutWhenUnconnected=off
  wires:
  lBuf/1 -> External Suspension Forces LEGACY/5(lBuf), Suspension Forces/5(lBuf)
  lStabi/1 -> External Suspension Forces LEGACY/4(lStabi), Suspension Forces/4(lStabi)
  vDamp/1 -> External Suspension Forces LEGACY/3(vDamp), Suspension Forces/3(vDamp)
  Tires/4(TireRR_Out) -> TireRR_Out/1
  Tires/3(TireRL_Out) -> TireRL_Out/1
  Tires/2(TireFR_Out) -> TireFR_Out/1
  Tires/1(TireFL_Out) -> TireFL_Out/1
  TireRR_In/1 -> Tires/5(TireRR_In)
  TireRL_In/1 -> Tires/4(TireRL_In)
  TireFR_In/1 -> Tires/3(TireFR_In)
  TireFL_In/1 -> Tires/2(TireFL_In)
  Sync_In/1 -> External Suspension Forces LEGACY/1(Sync_In), Tires/1(Sync_In), Vehicle Forces/1(Sync_In)
  Vehicle Forces/1(Sync_Out) -> Suspension Forces/1(Sync_In)
  Vehicle Forces/2(Car.Virtual) -> Car.Virtual/1
  Vehicle Forces/3(Car.Aero) -> Car.Aero/1
  Vehicle Forces/4(Car.Load) -> Car.Load/1
  lSpring/1 -> External Suspension Forces LEGACY/2(lSpring), Suspension Forces/2(lSpring)
  Suspension Forces/1(Sync_Out) -> Sync_Out/1

== system generic_IVS/CarMaker/IPG Vehicle/CarAndTrailer/Kinematics ==
  Sync_In : Inport
  Steer.IF : Inport  Port=2
  Kinematics : S-Function  FunctionName=CM_Sfun  Parameters='Kinematics'  SFunctionDeploymentMode=off  EnableBusSupport=off
  Terminator : Terminator
  Sync_Out : Outport  VectorParamsAs1DForOutWhenUnconnected=off
  TireFL_In : Outport  Port=2  VectorParamsAs1DForOutWhenUnconnected=off
  TireFR_In : Outport  Port=3  VectorParamsAs1DForOutWhenUnconnected=off
  TireRL_In : Outport  Port=4  VectorParamsAs1DForOutWhenUnconnected=off
  TireRR_In : Outport  Port=5  VectorParamsAs1DForOutWhenUnconnected=off
  lSpring : Outport  Port=6  VectorParamsAs1DForOutWhenUnconnected=off
  vDamp : Outport  Port=7  VectorParamsAs1DForOutWhenUnconnected=off
  lStabi : Outport  Port=8  VectorParamsAs1DForOutWhenUnconnected=off
  lBuf : Outport  Port=9  VectorParamsAs1DForOutWhenUnconnected=off
  wires:
  Kinematics/1 -> Sync_Out/1
  Kinematics/2 -> TireFL_In/1
  Kinematics/3 -> TireFR_In/1
  Kinematics/4 -> TireRL_In/1
  Kinematics/5 -> TireRR_In/1
  Kinematics/6 -> lSpring/1
  Kinematics/7 -> vDamp/1
  Kinematics/8 -> lStabi/1
  Kinematics/9 -> lBuf/1
  Kinematics/10 -> Terminator/1
  Sync_In/1 -> Kinematics/1
  Steer.IF/1 -> Kinematics/2

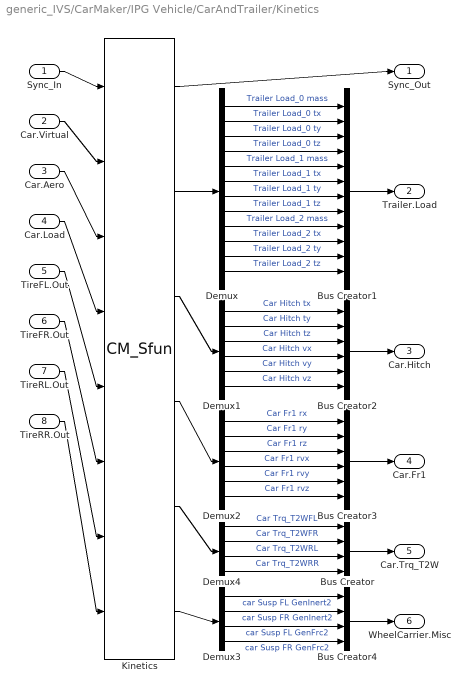
== system generic_IVS/CarMaker/IPG Vehicle/CarAndTrailer/Kinetics ==
  Sync_In : Inport
  Car.Virtual : Inport  Port=2
  Car.Aero : Inport  Port=3
  Car.Load : Inport  Port=4
  TireFL.Out : Inport  Port=5
  TireFR.Out : Inport  Port=6
  TireRL.Out : Inport  Port=7
  TireRR.Out : Inport  Port=8
  Bus Creator : BusCreator  Inputs=4
  Bus Creator1 : BusCreator  Inputs=12
  Bus Creator2 : BusCreator  Inputs=6
  Bus Creator3 : BusCreator  Inputs=6
  Bus Creator4 : BusCreator  Inputs=4
  Demux : Demux  Outputs=12
      settings: DisplayOption=none
  Demux1 : Demux  Outputs=6
      settings: DisplayOption=none
  Demux2 : Demux  Outputs=6
      settings: DisplayOption=none
  Demux3 : Demux
      settings: DisplayOption=none
  Demux4 : Demux
      settings: DisplayOption=none
  Kinetics : S-Function  FunctionName=CM_Sfun  Parameters='Kinetics'  SFunctionDeploymentMode=off  EnableBusSupport=off
  Sync_Out : Outport  VectorParamsAs1DForOutWhenUnconnected=off
  Trailer.Load : Outport  Port=2  VectorParamsAs1DForOutWhenUnconnected=off
  Car.Hitch : Outport  Port=3  VectorParamsAs1DForOutWhenUnconnected=off
  Car.Fr1 : Outport  Port=4  VectorParamsAs1DForOutWhenUnconnected=off
  Car.Trq_T2W : Outport  Port=5  VectorParamsAs1DForOutWhenUnconnected=off
  WheelCarrier.Misc : Outport  Port=6  VectorParamsAs1DForOutWhenUnconnected=off
  wires:
  Bus Creator1/1 -> Trailer.Load/1
  Demux/1 -> Bus Creator1/1  "Trailer Load_0 mass"
  Demux/2 -> Bus Creator1/2  "Trailer Load_0 tx"
  Demux/3 -> Bus Creator1/3  "Trailer Load_0 ty"
  Demux/4 -> Bus Creator1/4  "Trailer Load_0 tz"
  Demux/5 -> Bus Creator1/5  "Trailer Load_1 mass"
  Demux/6 -> Bus Creator1/6  "Trailer Load_1 tx"
  Demux/7 -> Bus Creator1/7  "Trailer Load_1 ty"
  Demux/8 -> Bus Creator1/8  "Trailer Load_1 tz"
  Demux/9 -> Bus Creator1/9  "Trailer Load_2 mass"
  Demux/10 -> Bus Creator1/10  "Trailer Load_2 tx"
  Demux/11 -> Bus Creator1/11  "Trailer Load_2 ty"
  Demux/12 -> Bus Creator1/12  "Trailer Load_2 tz"
  Demux1/1 -> Bus Creator2/1  "Car Hitch tx"
  Demux1/2 -> Bus Creator2/2  "Car Hitch ty"
  Demux1/3 -> Bus Creator2/3  "Car Hitch tz"
  Demux1/4 -> Bus Creator2/4  "Car Hitch vx"
  Demux1/5 -> Bus Creator2/5  "Car Hitch vy"
  Demux1/6 -> Bus Creator2/6  "Car Hitch vz"
  Bus Creator2/1 -> Car.Hitch/1
  Demux2/1 -> Bus Creator3/1  "Car Fr1 rx"
  Demux2/2 -> Bus Creator3/2  "Car Fr1 ry"
  Demux2/3 -> Bus Creator3/3  "Car Fr1 rz"
  Demux2/4 -> Bus Creator3/4  "Car Fr1 rvx"
  Demux2/5 -> Bus Creator3/5  "Car Fr1 rvy"
  Demux2/6 -> Bus Creator3/6  "Car Fr1 rvz"
  Bus Creator3/1 -> Car.Fr1/1
  Demux3/1 -> Bus Creator4/1  "car Susp FL GenInert2"
  Demux3/2 -> Bus Creator4/2  "car Susp FR GenInert2"
  Demux3/3 -> Bus Creator4/3  "car Susp FL GenFrc2"
  Demux3/4 -> Bus Creator4/4  "car Susp FR GenFrc2"
  Bus Creator4/1 -> WheelCarrier.Misc/1
  Bus Creator/1 -> Car.Trq_T2W/1
  Demux4/4 -> Bus Creator/4  "Car Trq_T2WRR"
  Demux4/3 -> Bus Creator/3  "Car Trq_T2WRL"
  Demux4/2 -> Bus Creator/2  "Car Trq_T2WFR"
  Demux4/1 -> Bus Creator/1  "Car Trq_T2WFL"
  Kinetics/1 -> Sync_Out/1
  Kinetics/2 -> Demux/1
  Kinetics/3 -> Demux1/1
  Kinetics/4 -> Demux2/1
  Kinetics/5 -> Demux4/1
  Kinetics/6 -> Demux3/1
  Sync_In/1 -> Kinetics/1
  Car.Virtual/1 -> Kinetics/2
  Car.Aero/1 -> Kinetics/3
  Car.Load/1 -> Kinetics/4
  TireFL.Out/1 -> Kinetics/5
  TireFR.Out/1 -> Kinetics/6
  TireRL.Out/1 -> Kinetics/7
  TireRR.Out/1 -> Kinetics/8

== system generic_IVS/CarMaker/IPG Vehicle/CarAndTrailer/Steering ==
  note: When replacing the entire steering system,
      | be sure to disable the IPG steering model by using the steering
      | model 'Model Manager off' in the vehicle GUI.
  Sync_In : Inport
  VhclCtrl.Steering : Inport  Port=2
  Bus Creator1 : BusCreator  Inputs=16
  Bus Creator2 : BusCreator  Inputs=5
  Demux : Demux  Outputs=21
      settings: DisplayOption=none
  Steering : S-Function  FunctionName=CM_Sfun  Parameters='Steering'  SFunctionDeploymentMode=off  EnableBusSupport=off
  Terminator : Terminator
  Sync_Out : Outport  VectorParamsAs1DForOutWhenUnconnected=off
  Steer.IF : Outport  Port=2  VectorParamsAs1DForOutWhenUnconnected=off
  wires:
  Demux/21 -> Bus Creator2/5  "Steering IF R Inert"
  Demux/20 -> Bus Creator2/4  "Steering IF R Frc"
  Demux/19 -> Bus Creator2/3  "Steering IF L Inert"
  Demux/18 -> Bus Creator2/2  "Steering IF L Frc"
  Demux/17 -> Bus Creator2/1  "Steering IF SteerByTrq"
  Demux/16 -> Bus Creator1/16  "Steering IF R iSteer2q"
  Demux/15 -> Bus Creator1/15  "Steering IF R qpp"
  Demux/14 -> Bus Creator1/14  "Steering IF R qp"
  Demux/13 -> Bus Creator1/13  "Steering IF R q"
  Demux/12 -> Bus Creator1/12  "Steering IF L iSteer2q"
  Demux/11 -> Bus Creator1/11  "Steering IF L qpp"
  Demux/10 -> Bus Creator1/10  "Steering IF L qp"
  Demux/9 -> Bus Creator1/9  "Steering IF L q"
  Demux/8 -> Bus Creator1/8  "Steering IF AssistTrqPin"
  Demux/7 -> Bus Creator1/7  "Steering IF AssistTrqCol"
  Demux/6 -> Bus Creator1/6  "Steering IF AssistFrc"
  Demux/5 -> Bus Creator1/5  "Steering IF TrqStatic"
  Demux/4 -> Bus Creator1/4  "Steering IF Trq"
  Demux/3 -> Bus Creator1/3  "Steering IF AngAcc"
  Demux/2 -> Bus Creator1/2  "Steering IF AngVel"
  Demux/1 -> Bus Creator1/1  "Steering IF Ang"
  Bus Creator1/1 -> Steer.IF/1
  Steering/2 -> Demux/1
  Bus Creator2/1 -> Terminator/1  "Steer IF (in)"
  VhclCtrl.Steering/1 -> Steering/2
  Steering/1 -> Sync_Out/1
  Sync_In/1 -> Steering/1

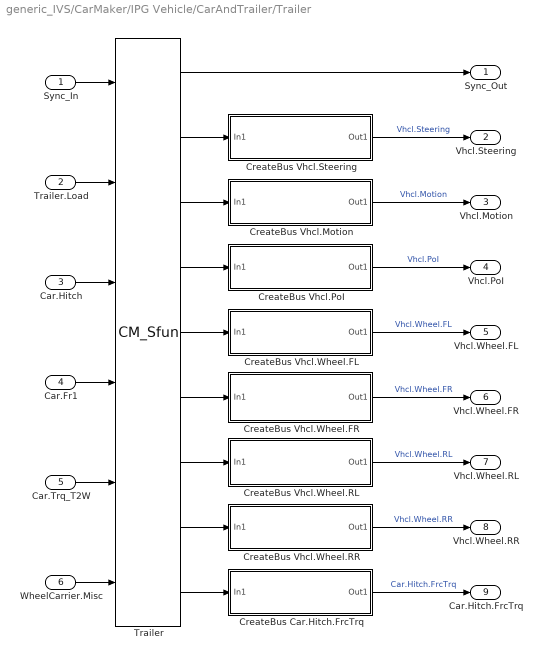
== system generic_IVS/CarMaker/IPG Vehicle/CarAndTrailer/Trailer ==
  Sync_In : Inport
  Trailer.Load : Inport  Port=2
  Car.Hitch : Inport  Port=3
  Car.Fr1 : Inport  Port=4
  Car.Trq_T2W : Inport  Port=5
  WheelCarrier.Misc : Inport  Port=6
  CreateBus Car.Hitch.FrcTrq : Subsystem
  CreateBus Vhcl.Motion : Subsystem
  CreateBus Vhcl.PoI : Subsystem
  CreateBus Vhcl.Steering : Subsystem
  CreateBus Vhcl.Wheel.FL : Subsystem
  CreateBus Vhcl.Wheel.FR : Subsystem
  CreateBus Vhcl.Wheel.RL : Subsystem
  CreateBus Vhcl.Wheel.RR : Subsystem
  Trailer : S-Function  FunctionName=CM_Sfun  Parameters='Trailer'  SFunctionDeploymentMode=off  EnableBusSupport=off
  Sync_Out : Outport  VectorParamsAs1DForOutWhenUnconnected=off
  Vhcl.Steering : Outport  Port=2  VectorParamsAs1DForOutWhenUnconnected=off
  Vhcl.Motion : Outport  Port=3  VectorParamsAs1DForOutWhenUnconnected=off
  Vhcl.PoI : Outport  Port=4  VectorParamsAs1DForOutWhenUnconnected=off
  Vhcl.Wheel.FL : Outport  Port=5  VectorParamsAs1DForOutWhenUnconnected=off
  Vhcl.Wheel.FR : Outport  Port=6  VectorParamsAs1DForOutWhenUnconnected=off
  Vhcl.Wheel.RL : Outport  Port=7  VectorParamsAs1DForOutWhenUnconnected=off
  Vhcl.Wheel.RR : Outport  Port=8  VectorParamsAs1DForOutWhenUnconnected=off
  Car.Hitch.FrcTrq : Outport  Port=9  VectorParamsAs1DForOutWhenUnconnected=off
  wires:
  Trailer/2 -> CreateBus Vhcl.Steering/1(In1)
  CreateBus Vhcl.Steering/1(Out1) -> Vhcl.Steering/1  "Vhcl.Steering"
  Trailer/3 -> CreateBus Vhcl.Motion/1(In1)
  Trailer/4 -> CreateBus Vhcl.PoI/1(In1)
  Trailer/5 -> CreateBus Vhcl.Wheel.FL/1(In1)
  Trailer/6 -> CreateBus Vhcl.Wheel.FR/1(In1)
  Trailer/7 -> CreateBus Vhcl.Wheel.RL/1(In1)
  Trailer/9 -> CreateBus Car.Hitch.FrcTrq/1(In1)
  Trailer/8 -> CreateBus Vhcl.Wheel.RR/1(In1)
  CreateBus Vhcl.Wheel.RR/1(Out1) -> Vhcl.Wheel.RR/1  "Vhcl.Wheel.RR"
  CreateBus Vhcl.Wheel.RL/1(Out1) -> Vhcl.Wheel.RL/1  "Vhcl.Wheel.RL"
  CreateBus Vhcl.Wheel.FR/1(Out1) -> Vhcl.Wheel.FR/1  "Vhcl.Wheel.FR"
  CreateBus Vhcl.Wheel.FL/1(Out1) -> Vhcl.Wheel.FL/1  "Vhcl.Wheel.FL"
  CreateBus Vhcl.PoI/1(Out1) -> Vhcl.PoI/1  "Vhcl.PoI"
  CreateBus Vhcl.Motion/1(Out1) -> Vhcl.Motion/1  "Vhcl.Motion"
  Car.Trq_T2W/1 -> Trailer/5
  WheelCarrier.Misc/1 -> Trailer/6
  CreateBus Car.Hitch.FrcTrq/1(Out1) -> Car.Hitch.FrcTrq/1  "Car.Hitch.FrcTrq"
  Car.Fr1/1 -> Trailer/4
  Car.Hitch/1 -> Trailer/3
  Trailer.Load/1 -> Trailer/2
  Trailer/1 -> Sync_Out/1
  Sync_In/1 -> Trailer/1

== system generic_IVS/CarMaker/IPG Vehicle/CarAndTrailer/CarAndTrailerUpd/CreateBus Brake.IF.In ==
  In : Inport
  BusCreator : BusCreator  Inputs=9
  Demux : Demux  Outputs=9
      settings: DisplayOption=none
  Out : Outport  VectorParamsAs1DForOutWhenUnconnected=off
  wires:
  Demux/9 -> BusCreator/9  "Brake IF Trq_Reg RR"
  Demux/8 -> BusCreator/8  "Brake IF Trq_Reg RL"
  Demux/7 -> BusCreator/7  "Brake IF Trq_Reg FR"
  Demux/6 -> BusCreator/6  "Brake IF Trq_Reg FL"
  Demux/5 -> BusCreator/5  "Brake IF Trq_Reg_max RR"
  Demux/4 -> BusCreator/4  "Brake IF Trq_Reg_max RL"
  Demux/3 -> BusCreator/3  "Brake IF Trq_Reg_max FR"
  Demux/2 -> BusCreator/2  "Brake IF Trq_Reg_max FL"
  Demux/1 -> BusCreator/1  "Brake IF T_env"
  BusCreator/1 -> Out/1
  In/1 -> Demux/1

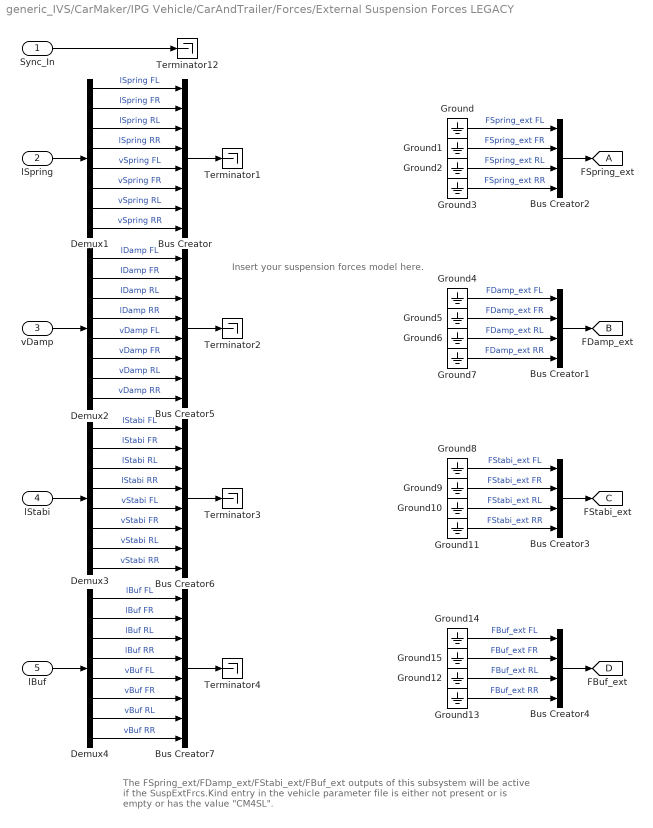
== system generic_IVS/CarMaker/IPG Vehicle/CarAndTrailer/Forces/External Suspension Forces LEGACY ==
  note: The FSpring_ext/FDamp_ext/FStabi_ext/FBuf_ext outputs of this subsystem will be
      | active if the SuspExtFrcs.Kind entry in the vehicle parameter file
      | is either not present or is empty or has the value "CM4SL".
  note: Insert your suspension forces model here.
  Sync_In : Inport
  lSpring : Inport  Port=2
  vDamp : Inport  Port=3
  lStabi : Inport  Port=4
  lBuf : Inport  Port=5
  Bus Creator{,5..7} (4 alike) : BusCreator  Inputs=8
  Bus Creator{1..4} (4 alike) : BusCreator  Inputs=4
  Demux{1..4} (4 alike) : Demux  Outputs=8
      settings: DisplayOption=none
  FSpring_ext : Goto  TagVisibility=global
  Ground{,1..15} (16 alike) : Ground
  Terminator{1..4,12} (5 alike) : Terminator
  tag scope: B=global, C=global, D=global
  wires:
  Bus Creator7/1 -> Terminator4/1
  Bus Creator6/1 -> Terminator3/1
  Bus Creator5/1 -> Terminator2/1
  Bus Creator/1 -> Terminator1/1
  Demux4/8 -> Bus Creator7/8  "vBuf RR"
  Demux4/7 -> Bus Creator7/7  "vBuf RL"
  Demux4/6 -> Bus Creator7/6  "vBuf FR"
  Demux4/5 -> Bus Creator7/5  "vBuf FL"
  Demux3/8 -> Bus Creator6/8  "vStabi RR"
  Demux3/7 -> Bus Creator6/7  "vStabi RL"
  Demux3/6 -> Bus Creator6/6  "vStabi FR"
  Demux3/5 -> Bus Creator6/5  "vStabi FL"
  Demux2/8 -> Bus Creator5/8  "vDamp RR"
  Demux2/7 -> Bus Creator5/7  "vDamp RL"
  Demux2/6 -> Bus Creator5/6  "vDamp FR"
  Demux2/5 -> Bus Creator5/5  "vDamp FL"
  Demux1/8 -> Bus Creator/8  "vSpring RR"
  Demux1/7 -> Bus Creator/7  "vSpring RL"
  Demux1/6 -> Bus Creator/6  "vSpring FR"
  Demux1/5 -> Bus Creator/5  "vSpring FL"
  Demux2/4 -> Bus Creator5/4  "lDamp RR"
  Demux2/3 -> Bus Creator5/3  "lDamp RL"
  Demux2/2 -> Bus Creator5/2  "lDamp FR"
  Demux2/1 -> Bus Creator5/1  "lDamp FL"
  Demux1/4 -> Bus Creator/4  "lSpring RR"
  Demux1/3 -> Bus Creator/3  "lSpring RL"
  Demux1/2 -> Bus Creator/2  "lSpring FR"
  Demux1/1 -> Bus Creator/1  "lSpring FL"
  Demux3/4 -> Bus Creator6/4  "lStabi RR"
  Demux3/3 -> Bus Creator6/3  "lStabi RL"
  Demux3/2 -> Bus Creator6/2  "lStabi FR"
  Demux3/1 -> Bus Creator6/1  "lStabi FL"
  lStabi/1 -> Demux3/1
  vDamp/1 -> Demux2/1
  lSpring/1 -> Demux1/1
  Demux4/4 -> Bus Creator7/4  "lBuf RR"
  Demux4/3 -> Bus Creator7/3  "lBuf RL"
  Demux4/2 -> Bus Creator7/2  "lBuf FR"
  Demux4/1 -> Bus Creator7/1  "lBuf FL"
  lBuf/1 -> Demux4/1
  Ground14/1 -> Bus Creator4/1  "FBuf_ext FL"
  Ground15/1 -> Bus Creator4/2  "FBuf_ext FR"
  Ground12/1 -> Bus Creator4/3  "FBuf_ext RL"
  Ground13/1 -> Bus Creator4/4  "FBuf_ext RR"
  Sync_In/1 -> Terminator12/1
  Ground/1 -> Bus Creator2/1  "FSpring_ext FL"
  Ground1/1 -> Bus Creator2/2  "FSpring_ext FR"
  Ground2/1 -> Bus Creator2/3  "FSpring_ext RL"
  Ground3/1 -> Bus Creator2/4  "FSpring_ext RR"
  Ground4/1 -> Bus Creator1/1  "FDamp_ext FL"
  Ground5/1 -> Bus Creator1/2  "FDamp_ext FR"
  Ground6/1 -> Bus Creator1/3  "FDamp_ext RL"
  Ground7/1 -> Bus Creator1/4  "FDamp_ext RR"
  Ground8/1 -> Bus Creator3/1  "FStabi_ext FL"
  Ground9/1 -> Bus Creator3/2  "FStabi_ext FR"
  Ground10/1 -> Bus Creator3/3  "FStabi_ext RL"
  Ground11/1 -> Bus Creator3/4  "FStabi_ext RR"
  Bus Creator2/1 -> FSpring_ext/1
  Bus Creator1/1 -> [B]
  Bus Creator3/1 -> [C]
  Bus Creator4/1 -> [D]

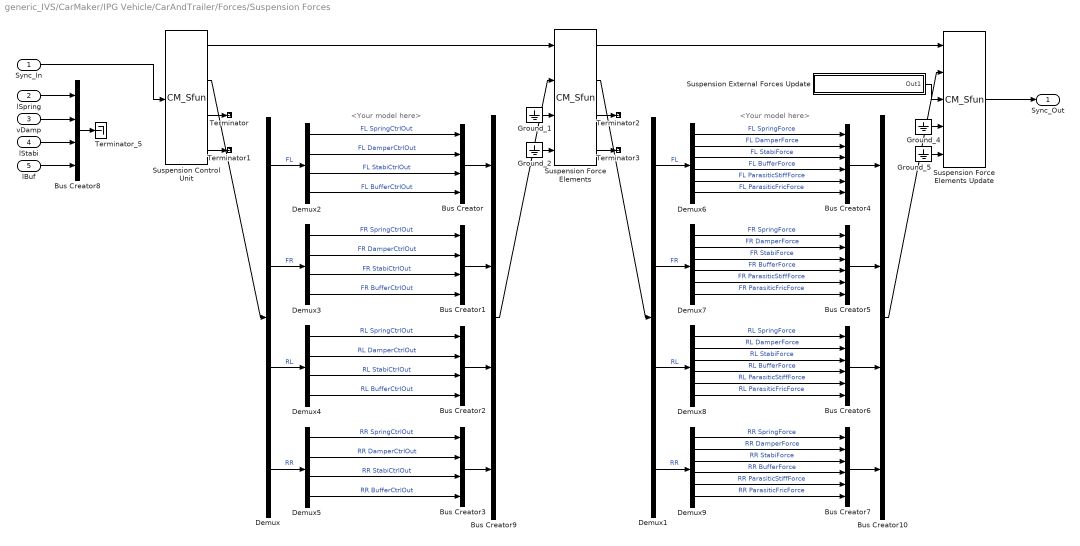
== system generic_IVS/CarMaker/IPG Vehicle/CarAndTrailer/Forces/Suspension Forces ==
  note: <Your model here>
  note: <Your model here>
  Sync_In : Inport
  lSpring : Inport  Port=2
  vDamp : Inport  Port=3
  lStabi : Inport  Port=4
  lBuf : Inport  Port=5
  Bus Creator{,1..3,8..10} (7 alike) : BusCreator  Inputs=4
  Bus Creator{4..7} (4 alike) : BusCreator  Inputs=6
  Demux{,1..5} (6 alike) : Demux
  Demux{6..9} (4 alike) : Demux  Outputs=6
  Ground_{1..2,4..5} (4 alike) : Ground
  Suspension Control Unit : S-Function  FunctionName=CM_Sfun  Parameters='ForcesSuspControl'  SFunctionDeploymentMode=off  EnableBusSupport=off
  Suspension External Forces Update : Subsystem
  Suspension Force Elements : S-Function  FunctionName=CM_Sfun  Parameters='ForcesSusp'  SFunctionDeploymentMode=off  EnableBusSupport=off
  Suspension Force Elements Update : S-Function  FunctionName=CM_Sfun  Parameters='ForcesSuspUpd'  SFunctionDeploymentMode=off  EnableBusSupport=off
  Terminator{,1..3} (4 alike) : Terminator
  Terminator_5 : Terminator
  Sync_Out : Outport  VectorParamsAs1DForOutWhenUnconnected=off
  wires:
  vDamp/1 -> Bus Creator8/2
  lStabi/1 -> Bus Creator8/3
  lBuf/1 -> Bus Creator8/4
  lSpring/1 -> Bus Creator8/1
  Bus Creator4/1 -> Bus Creator10/1
  Bus Creator5/1 -> Bus Creator10/2
  Bus Creator6/1 -> Bus Creator10/3
  Bus Creator7/1 -> Bus Creator10/4
  Demux6/1 -> Bus Creator4/1  "FL SpringForce"
  Demux9/1 -> Bus Creator7/1  "RR SpringForce"
  Demux9/2 -> Bus Creator7/2  "RR DamperForce"
  Demux9/3 -> Bus Creator7/3  "RR StabiForce"
  Demux9/4 -> Bus Creator7/4  "RR BufferForce"
  Demux9/5 -> Bus Creator7/5  "RR ParasiticStiffForce"
  Demux9/6 -> Bus Creator7/6  "RR ParasiticFricForce"
  Demux8/1 -> Bus Creator6/1  "RL SpringForce"
  Demux8/2 -> Bus Creator6/2  "RL DamperForce"
  Demux8/4 -> Bus Creator6/4  "RL BufferForce"
  Demux8/5 -> Bus Creator6/5  "RL ParasiticStiffForce"
  Demux8/6 -> Bus Creator6/6  "RL ParasiticFricForce"
  Demux8/3 -> Bus Creator6/3  "RL StabiForce"
  Demux7/1 -> Bus Creator5/1  "FR SpringForce"
  Demux7/2 -> Bus Creator5/2  "FR DamperForce"
  Demux7/3 -> Bus Creator5/3  "FR StabiForce"
  Demux7/4 -> Bus Creator5/4  "FR BufferForce"
  Demux7/5 -> Bus Creator5/5  "FR ParasiticStiffForce"
  Demux7/6 -> Bus Creator5/6  "FR ParasiticFricForce"
  Demux6/2 -> Bus Creator4/2  "FL DamperForce"
  Demux6/3 -> Bus Creator4/3  "FL StabiForce"
  Demux6/4 -> Bus Creator4/4  "FL BufferForce"
  Demux6/5 -> Bus Creator4/5  "FL ParasiticStiffForce"
  Demux6/6 -> Bus Creator4/6  "FL ParasiticFricForce"
  Demux/1 -> Demux2/1  "FL"
  Bus Creator1/1 -> Bus Creator9/2
  Demux/2 -> Demux3/1  "FR"
  Bus Creator2/1 -> Bus Creator9/3
  Demux/3 -> Demux4/1  "RL"
  Bus Creator3/1 -> Bus Creator9/4
  Demux2/1 -> Bus Creator/1  "FL SpringCtrlOut"
  Demux/4 -> Demux5/1  "RR"
  Demux5/1 -> Bus Creator3/1  "RR SpringCtrlOut"
  Demux5/2 -> Bus Creator3/2  "RR DamperCtrlOut"
  Demux5/3 -> Bus Creator3/3  "RR StabiCtrlOut"
  Demux5/4 -> Bus Creator3/4  "RR BufferCtrlOut"
  Demux4/1 -> Bus Creator2/1  "RL SpringCtrlOut"
  Demux4/2 -> Bus Creator2/2  "RL DamperCtrlOut"
  Demux4/4 -> Bus Creator2/4  "RL BufferCtrlOut"
  Demux4/3 -> Bus Creator2/3  "RL StabiCtrlOut"
  Demux3/1 -> Bus Creator1/1  "FR SpringCtrlOut"
  Demux3/2 -> Bus Creator1/2  "FR DamperCtrlOut"
  Demux3/3 -> Bus Creator1/3  "FR StabiCtrlOut"
  Demux3/4 -> Bus Creator1/4  "FR BufferCtrlOut"
  Demux2/2 -> Bus Creator/2  "FL DamperCtrlOut"
  Demux2/3 -> Bus Creator/3  "FL StabiCtrlOut"
  Demux2/4 -> Bus Creator/4  "FL BufferCtrlOut"
  Bus Creator/1 -> Bus Creator9/1
  Demux1/1 -> Demux6/1  "FL"
  Demux1/2 -> Demux7/1  "FR"
  Demux1/3 -> Demux8/1  "RL"
  Demux1/4 -> Demux9/1  "RR"
  Suspension Control Unit/2 -> Demux/1
  Suspension Control Unit/3 -> Terminator/1
  Suspension Control Unit/4 -> Terminator1/1
  Sync_In/1 -> Suspension Control Unit/1
  Suspension Force Elements/2 -> Demux1/1
  Suspension Force Elements/3 -> Terminator2/1
  Suspension Force Elements/4 -> Terminator3/1
  Suspension Control Unit/1 -> Suspension Force Elements/1
  Bus Creator9/1 -> Suspension Force Elements/2
  Bus Creator8/1 -> Terminator_5/1
  Ground_1/1 -> Suspension Force Elements/3
  Ground_2/1 -> Suspension Force Elements/4
  Suspension Force Elements Update/1 -> Sync_Out/1
  Suspension Force Elements/1 -> Suspension Force Elements Update/1
  Bus Creator10/1 -> Suspension Force Elements Update/2
  Ground_4/1 -> Suspension Force Elements Update/4
  Ground_5/1 -> Suspension Force Elements Update/5
  Suspension External Forces Update/1(Out1) -> Suspension Force Elements Update/3
